simulink model "tanque"  (R2016b)
settings: Solver=ode15s  StartTime=0.0  StopTime=Inf  RelTol=1e-3  EnableMultiTasking=on
libraries: simulink_extras x3
(part 2 of 2)

== system tanque/B 111 ==
  note: Exaustor
  Sinal de entrada : Inport
  Sinal de saída : Outport
  wires:
  Sinal de entrada/1 -> Sinal de saída/1

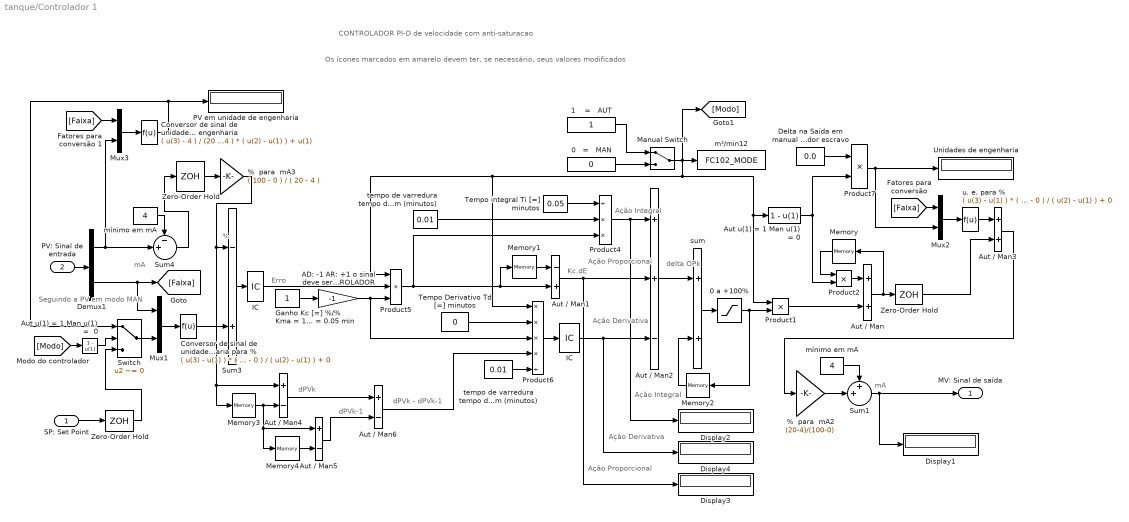
== system tanque/Controlador 1 ==
  note: Ação
      | Derivativa
  note: dPVk - dPVk-1
  note: dPVk
  note: dPVk-1
  note: delta
      | OPk
  note: Ação
      | Integral
  note: Ação
      | Proporcional
  note: Kc.dE
  note: %
  note: mA
  note: CONTROLADOR PI-D de velocidade com anti-saturacao
  note: Os ícones marcados em amarelo devem ter, se necessário, seus valores modificados
  note: Erro
  note: mA
  note: Ação
      | Integral
  note: Ação
      | Derivativa
  note: Ação
      | Proporcional
  note: Seguindo a PV
      | em modo MAN
  SP: Set Point : Inport
  PV: Sinal de entrada : Inport  Port=2
  "  1    =   AUT" : Constant
  " IC" : InitialCondition  Value=0
  %  para  mA2 : Gain  Gain=(20-4)/(100-0)  SaturateOnIntegerOverflow=on  OutDataTypeStr=Inherit: Same as input  ParamDataTypeStr=Inherit: Same as input
  %  para  mA3 : Gain  Gain=( 100 - 0 ) / ( 20 - 4 )  SaturateOnIntegerOverflow=on  OutDataTypeStr=Inherit: Same as input  ParamDataTypeStr=Inherit: Same as input
  0   =   MAN : Constant  Value=0
  0 a +100% : Saturate  UpperLimit=100  LowerLimit=0  LinearizeAsGain=off
  "AD: -1 AR: +1 o sinal deve ser modificado para a correta  AÇÃO  DO  CONTROLADOR " : Gain  Gain=-1  SaturateOnIntegerOverflow=on  OutDataTypeStr=Inherit: Same as input  ParamDataTypeStr=Inherit: Same as input
  Aut / Man : Sum  SaturateOnIntegerOverflow=on  InputSameDT=on  OutDataTypeStr=Inherit: Same as first input
  Aut / Man1 : Sum  Inputs=-+  SaturateOnIntegerOverflow=on  InputSameDT=on  OutDataTypeStr=Inherit: Same as first input
  Aut / Man2 : Sum  Inputs=++-  SaturateOnIntegerOverflow=on  InputSameDT=on  OutDataTypeStr=Inherit: Same as first input
  Aut / Man3 : Sum  SaturateOnIntegerOverflow=on  InputSameDT=on  OutDataTypeStr=Inherit: Same as first input
  Aut / Man4 : Sum  Inputs=+-  SaturateOnIntegerOverflow=on  InputSameDT=on  OutDataTypeStr=Inherit: Same as first input
  Aut / Man5 : Sum  Inputs=+-  SaturateOnIntegerOverflow=on  InputSameDT=on  OutDataTypeStr=Inherit: Same as first input
  Aut / Man6 : Sum  Inputs=+-  SaturateOnIntegerOverflow=on  InputSameDT=on  OutDataTypeStr=Inherit: Same as first input
  Aut u(1) = 1 Man u(1) =  0 : Fcn  Expr=1 - u(1)
  Aut u(1) = 1 Man u(1) = 0 : Fcn  Expr=1 - u(1)
  Conversor de sinal de unidades de engenharia para % : Fcn  Expr=( u(3) - u(1) ) * ( 100 - 0 ) / ( u(2) - u(1) ) + 0
  Conversor de sinal de unidades de  mA  para engenharia : Fcn  Expr=( u(3) - 4 ) / (20 - 4 ) * ( u(2) - u(1) ) + u(1)
  Delta na Saída em manual do controlador [=] unidades de engenharia do SP do controlador escravo : Constant  Value=0.0
  Demux1 : Demux  Outputs=[ 1 2 ]
  Display{1..4} (4 alike) : Display
  Ganho Kc [=] %/% Kma = 1 mA/mA Lambda = 0.05 min : Constant
  IC : InitialCondition  Value=0
  Manual Switch : ManualSwitch
  Memory{,2..4} (4 alike) : Memory  X0=50  InheritSampleTime=on
  Memory1 : Memory  InheritSampleTime=on
  Mux1 : Mux  Inputs=[ 2 1 ]
  Mux2 : Mux  Inputs=[ 2 1 ]
  Mux3 : Mux  Inputs=[ 2 1 ]
  PV em unidade de engenharia : Display
  Product1 : Product  SaturateOnIntegerOverflow=on  RndMeth=Zero  InputSameDT=on  OutDataTypeStr=Inherit: Same as first input
  Product2 : Product  SaturateOnIntegerOverflow=on  RndMeth=Zero  InputSameDT=on  OutDataTypeStr=Inherit: Same as first input
  Product4 : Product  Inputs=/**  SaturateOnIntegerOverflow=on  RndMeth=Zero  InputSameDT=on  OutDataTypeStr=Inherit: Same as first input
  Product5 : Product  Inputs=3  SaturateOnIntegerOverflow=on  RndMeth=Zero  InputSameDT=on  OutDataTypeStr=Inherit: Same as first input
  Product6 : Product  Inputs=****/  SaturateOnIntegerOverflow=on  RndMeth=Zero  InputSameDT=on  OutDataTypeStr=Inherit: Same as first input
  Product7 : Product  SaturateOnIntegerOverflow=on  RndMeth=Zero  InputSameDT=on  OutDataTypeStr=Inherit: Same as first input
  Sum1 : Sum  Inputs=++|  SaturateOnIntegerOverflow=on  InputSameDT=on  OutDataTypeStr=Inherit: Same as first input
  Sum3 : Sum  Inputs=-+  SaturateOnIntegerOverflow=on  InputSameDT=on  OutDataTypeStr=Inherit: Same as first input
  Sum4 : Sum  Inputs=-+|  SaturateOnIntegerOverflow=on  InputSameDT=on  OutDataTypeStr=Inherit: Same as first input
  Switch : Switch  Criteria=u2 ~= 0  RndMeth=Nearest  SaturateOnIntegerOverflow=on
  Tempo Derivativo Td [=] minutos : Constant  Value=0
  Tempo integral Ti [=] minutos : Constant  Value=0.05
  Unidades de engenharia : Display
  Zero-Order Hold : ZeroOrderHold  SampleTime=0.01
  "Zero-Order Hold " : ZeroOrderHold  SampleTime=0.01
  "Zero-Order Hold " : ZeroOrderHold  SampleTime=0.01
  m³/min12 : ToWorkspace  VariableName=FC102_MODE  SampleTime=-1
      settings: Decimation=10
  mínimo em mA : Constant  Value=4
  "mínimo em mA " : Constant  Value=4
  sum : Sum  SaturateOnIntegerOverflow=on  InputSameDT=on  OutDataTypeStr=Inherit: Same as first input
  tempo de varredura tempo de amostragem (minutos) : Constant  Value=0.01
  "tempo de varredura tempo de amostragem (minutos) " : Constant  Value=0.01
  u. e. para % : Fcn  Expr=( u(3) - u(1) ) * ( 100 - 0 ) / ( u(2) - u(1) ) + 0
  MV: Sinal de saída : Outport
  wires:
  "AD: -1 AR: +1 o sinal deve ser modificado para a correta  AÇÃO  DO  CONTROLADOR "/1 -> Product5/3, Product6/3
  " IC"/1 -> Aut / Man2/3, Display4/1
  "tempo de varredura tempo de amostragem (minutos) "/1 -> Product6/5
  Aut / Man5/1 -> Aut / Man6/2
  Aut / Man4/1 -> Aut / Man6/1
  Conversor de sinal de unidades de engenharia para %/1 -> Sum3/2
  Product6/1 -> " IC"/1
  Tempo Derivativo Td [=] minutos/1 -> Product6/2
  Aut / Man6/1 -> Product6/4
  Memory4/1 -> Aut / Man5/2
  Memory3/1 -> Aut / Man4/2, Aut / Man5/1, Memory4/1
  Ganho Kc [=] %/% Kma = 1 mA/mA Lambda = 0.05 min/1 -> "AD: -1 AR: +1 o sinal deve ser modificado para a correta  AÇÃO  DO  CONTROLADOR "/1
  IC/1 -> Product5/2
  0 a +100%/1 -> Product1/2, Memory2/1
  Memory2/1 -> sum/2
  sum/1 -> 0 a +100%/1
  Aut / Man2/1 -> sum/1
  Aut / Man1/1 -> Aut / Man2/2, Display3/1
  Product4/1 -> Aut / Man2/1, Display2/1
  Memory1/1 -> Aut / Man1/1
  Memory/1 -> Product2/1
  Aut / Man/1 -> Memory/1, Zero-Order Hold/1
  Aut u(1) = 1 Man u(1) = 0/1 -> Product2/2, Product7/2
  Product2/1 -> Aut / Man/1
  Product1/1 -> Aut / Man/2
  Product5/1 -> Memory1/1, Aut / Man1/2, Product4/3
  Sum3/1 -> IC/1
  mínimo em mA/1 -> Sum4/1
  Demux1/1 -> Sum4/2, Mux3/2
  Mux1/1 -> Conversor de sinal de unidades de engenharia para %/1
  SP: Set Point/1 -> "Zero-Order Hold "/1
  PV: Sinal de entrada/1 -> Demux1/1
  "mínimo em mA "/1 -> Sum1/1
  Sum1/1 -> MV: Sinal de saída/1, Display1/1
  Sum4/1 -> "Zero-Order Hold "/1
  "Zero-Order Hold "/1 -> %  para  mA3/1
  %  para  mA3/1 -> Memory3/1, Aut / Man4/1, Sum3/1
  Manual Switch/1 -> Aut u(1) = 1 Man u(1) = 0/1, Product1/1, Product5/1, Product6/1, [Modo], m³/min12/1
  Delta na Saída em manual do controlador [=] unidades de engenharia do SP do controlador escravo/1 -> Product7/1
  Product7/1 -> Unidades de engenharia/1, Mux2/2
  Demux1/2 -> Mux1/1, [Faixa]
  "Zero-Order Hold "/1 -> Switch/3
  u. e. para %/1 -> Aut / Man3/1
  Zero-Order Hold/1 -> Aut / Man3/2
  Mux2/1 -> u. e. para %/1
  [Faixa] -> Mux2/1
  Aut / Man3/1 -> %  para  mA2/1
  %  para  mA2/1 -> Sum1/2
  "  1    =   AUT"/1 -> Manual Switch/1
  0   =   MAN/1 -> Manual Switch/2
  [Modo] -> Aut u(1) = 1 Man u(1) =  0/1
  Switch/1 -> Mux1/2
  Aut u(1) = 1 Man u(1) =  0/1 -> Switch/2
  Mux3/1 -> Conversor de sinal de unidades de  mA  para engenharia/1
  [Faixa] -> Mux3/1
  Conversor de sinal de unidades de  mA  para engenharia/1 -> Switch/1, PV em unidade de engenharia/1
  Tempo integral Ti [=] minutos/1 -> Product4/1
  tempo de varredura tempo de amostragem (minutos)/1 -> Product4/2

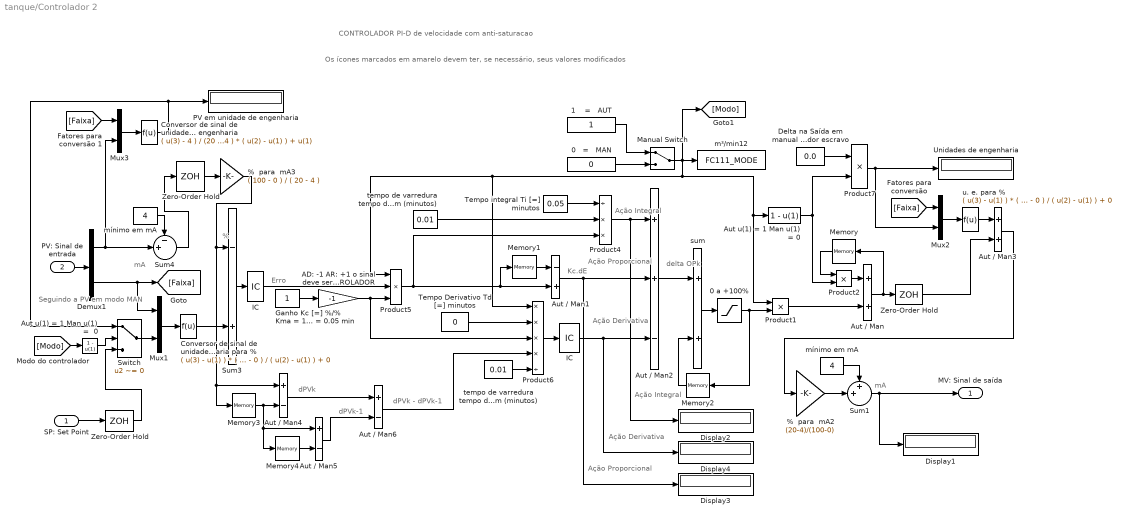
== system tanque/Controlador 2 ==
  note: Ação
      | Derivativa
  note: dPVk - dPVk-1
  note: dPVk
  note: dPVk-1
  note: delta
      | OPk
  note: Ação
      | Integral
  note: Ação
      | Proporcional
  note: Kc.dE
  note: %
  note: mA
  note: CONTROLADOR PI-D de velocidade com anti-saturacao
  note: Os ícones marcados em amarelo devem ter, se necessário, seus valores modificados
  note: Erro
  note: mA
  note: Ação
      | Integral
  note: Ação
      | Derivativa
  note: Ação
      | Proporcional
  note: Seguindo a PV
      | em modo MAN
  SP: Set Point : Inport
  PV: Sinal de entrada : Inport  Port=2
  "  1    =   AUT" : Constant
  " IC" : InitialCondition  Value=0
  %  para  mA2 : Gain  Gain=(20-4)/(100-0)  SaturateOnIntegerOverflow=on  OutDataTypeStr=Inherit: Same as input  ParamDataTypeStr=Inherit: Same as input
  %  para  mA3 : Gain  Gain=( 100 - 0 ) / ( 20 - 4 )  SaturateOnIntegerOverflow=on  OutDataTypeStr=Inherit: Same as input  ParamDataTypeStr=Inherit: Same as input
  0   =   MAN : Constant  Value=0
  0 a +100% : Saturate  UpperLimit=100  LowerLimit=0  LinearizeAsGain=off
  "AD: -1 AR: +1 o sinal deve ser modificado para a correta  AÇÃO  DO  CONTROLADOR " : Gain  Gain=-1  SaturateOnIntegerOverflow=on  OutDataTypeStr=Inherit: Same as input  ParamDataTypeStr=Inherit: Same as input
  Aut / Man : Sum  SaturateOnIntegerOverflow=on  InputSameDT=on  OutDataTypeStr=Inherit: Same as first input
  Aut / Man1 : Sum  Inputs=-+  SaturateOnIntegerOverflow=on  InputSameDT=on  OutDataTypeStr=Inherit: Same as first input
  Aut / Man2 : Sum  Inputs=++-  SaturateOnIntegerOverflow=on  InputSameDT=on  OutDataTypeStr=Inherit: Same as first input
  Aut / Man3 : Sum  SaturateOnIntegerOverflow=on  InputSameDT=on  OutDataTypeStr=Inherit: Same as first input
  Aut / Man4 : Sum  Inputs=+-  SaturateOnIntegerOverflow=on  InputSameDT=on  OutDataTypeStr=Inherit: Same as first input
  Aut / Man5 : Sum  Inputs=+-  SaturateOnIntegerOverflow=on  InputSameDT=on  OutDataTypeStr=Inherit: Same as first input
  Aut / Man6 : Sum  Inputs=+-  SaturateOnIntegerOverflow=on  InputSameDT=on  OutDataTypeStr=Inherit: Same as first input
  Aut u(1) = 1 Man u(1) =  0 : Fcn  Expr=1 - u(1)
  Aut u(1) = 1 Man u(1) = 0 : Fcn  Expr=1 - u(1)
  Conversor de sinal de unidades de engenharia para % : Fcn  Expr=( u(3) - u(1) ) * ( 100 - 0 ) / ( u(2) - u(1) ) + 0
  Conversor de sinal de unidades de  mA  para engenharia : Fcn  Expr=( u(3) - 4 ) / (20 - 4 ) * ( u(2) - u(1) ) + u(1)
  Delta na Saída em manual do controlador [=] unidades de engenharia do SP do controlador escravo : Constant  Value=0.0
  Demux1 : Demux  Outputs=[ 1 2 ]
  Display{1..4} (4 alike) : Display
  Ganho Kc [=] %/% Kma = 1 mA/mA Lambda = 0.05 min : Constant
  IC : InitialCondition  Value=0
  Manual Switch : ManualSwitch
  Memory{,2..4} (4 alike) : Memory  X0=50  InheritSampleTime=on
  Memory1 : Memory  InheritSampleTime=on
  Mux1 : Mux  Inputs=[ 2 1 ]
  Mux2 : Mux  Inputs=[ 2 1 ]
  Mux3 : Mux  Inputs=[ 2 1 ]
  PV em unidade de engenharia : Display
  Product1 : Product  SaturateOnIntegerOverflow=on  RndMeth=Zero  InputSameDT=on  OutDataTypeStr=Inherit: Same as first input
  Product2 : Product  SaturateOnIntegerOverflow=on  RndMeth=Zero  InputSameDT=on  OutDataTypeStr=Inherit: Same as first input
  Product4 : Product  Inputs=/**  SaturateOnIntegerOverflow=on  RndMeth=Zero  InputSameDT=on  OutDataTypeStr=Inherit: Same as first input
  Product5 : Product  Inputs=3  SaturateOnIntegerOverflow=on  RndMeth=Zero  InputSameDT=on  OutDataTypeStr=Inherit: Same as first input
  Product6 : Product  Inputs=****/  SaturateOnIntegerOverflow=on  RndMeth=Zero  InputSameDT=on  OutDataTypeStr=Inherit: Same as first input
  Product7 : Product  SaturateOnIntegerOverflow=on  RndMeth=Zero  InputSameDT=on  OutDataTypeStr=Inherit: Same as first input
  Sum1 : Sum  Inputs=++|  SaturateOnIntegerOverflow=on  InputSameDT=on  OutDataTypeStr=Inherit: Same as first input
  Sum3 : Sum  Inputs=-+  SaturateOnIntegerOverflow=on  InputSameDT=on  OutDataTypeStr=Inherit: Same as first input
  Sum4 : Sum  Inputs=-+|  SaturateOnIntegerOverflow=on  InputSameDT=on  OutDataTypeStr=Inherit: Same as first input
  Switch : Switch  Criteria=u2 ~= 0  RndMeth=Nearest  SaturateOnIntegerOverflow=on
  Tempo Derivativo Td [=] minutos : Constant  Value=0
  Tempo integral Ti [=] minutos : Constant  Value=0.05
  Unidades de engenharia : Display
  Zero-Order Hold : ZeroOrderHold  SampleTime=0.01
  "Zero-Order Hold " : ZeroOrderHold  SampleTime=0.01
  "Zero-Order Hold " : ZeroOrderHold  SampleTime=0.01
  m³/min12 : ToWorkspace  VariableName=FC111_MODE  SampleTime=-1
      settings: Decimation=10
  mínimo em mA : Constant  Value=4
  "mínimo em mA " : Constant  Value=4
  sum : Sum  SaturateOnIntegerOverflow=on  InputSameDT=on  OutDataTypeStr=Inherit: Same as first input
  tempo de varredura tempo de amostragem (minutos) : Constant  Value=0.01
  "tempo de varredura tempo de amostragem (minutos) " : Constant  Value=0.01
  u. e. para % : Fcn  Expr=( u(3) - u(1) ) * ( 100 - 0 ) / ( u(2) - u(1) ) + 0
  MV: Sinal de saída : Outport
  wires:
  "AD: -1 AR: +1 o sinal deve ser modificado para a correta  AÇÃO  DO  CONTROLADOR "/1 -> Product5/3, Product6/3
  " IC"/1 -> Aut / Man2/3, Display4/1
  "tempo de varredura tempo de amostragem (minutos) "/1 -> Product6/5
  Aut / Man5/1 -> Aut / Man6/2
  Aut / Man4/1 -> Aut / Man6/1
  Conversor de sinal de unidades de engenharia para %/1 -> Sum3/2
  Product6/1 -> " IC"/1
  Tempo Derivativo Td [=] minutos/1 -> Product6/2
  Aut / Man6/1 -> Product6/4
  Memory4/1 -> Aut / Man5/2
  Memory3/1 -> Aut / Man4/2, Aut / Man5/1, Memory4/1
  Ganho Kc [=] %/% Kma = 1 mA/mA Lambda = 0.05 min/1 -> "AD: -1 AR: +1 o sinal deve ser modificado para a correta  AÇÃO  DO  CONTROLADOR "/1
  IC/1 -> Product5/2
  0 a +100%/1 -> Product1/2, Memory2/1
  Memory2/1 -> sum/2
  sum/1 -> 0 a +100%/1
  Aut / Man2/1 -> sum/1
  Aut / Man1/1 -> Aut / Man2/2, Display3/1
  Product4/1 -> Aut / Man2/1, Display2/1
  Memory1/1 -> Aut / Man1/1
  Memory/1 -> Product2/1
  Aut / Man/1 -> Memory/1, Zero-Order Hold/1
  Aut u(1) = 1 Man u(1) = 0/1 -> Product2/2, Product7/2
  Product2/1 -> Aut / Man/1
  Product1/1 -> Aut / Man/2
  Product5/1 -> Memory1/1, Aut / Man1/2, Product4/3
  Sum3/1 -> IC/1
  mínimo em mA/1 -> Sum4/1
  Demux1/1 -> Sum4/2, Mux3/2
  Mux1/1 -> Conversor de sinal de unidades de engenharia para %/1
  SP: Set Point/1 -> "Zero-Order Hold "/1
  PV: Sinal de entrada/1 -> Demux1/1
  "mínimo em mA "/1 -> Sum1/1
  Sum1/1 -> MV: Sinal de saída/1, Display1/1
  Sum4/1 -> "Zero-Order Hold "/1
  "Zero-Order Hold "/1 -> %  para  mA3/1
  %  para  mA3/1 -> Memory3/1, Aut / Man4/1, Sum3/1
  Manual Switch/1 -> Aut u(1) = 1 Man u(1) = 0/1, Product1/1, Product5/1, Product6/1, [Modo], m³/min12/1
  Delta na Saída em manual do controlador [=] unidades de engenharia do SP do controlador escravo/1 -> Product7/1
  Product7/1 -> Unidades de engenharia/1, Mux2/2
  Demux1/2 -> Mux1/1, [Faixa]
  "Zero-Order Hold "/1 -> Switch/3
  u. e. para %/1 -> Aut / Man3/1
  Zero-Order Hold/1 -> Aut / Man3/2
  Mux2/1 -> u. e. para %/1
  [Faixa] -> Mux2/1
  Aut / Man3/1 -> %  para  mA2/1
  %  para  mA2/1 -> Sum1/2
  "  1    =   AUT"/1 -> Manual Switch/1
  0   =   MAN/1 -> Manual Switch/2
  [Modo] -> Aut u(1) = 1 Man u(1) =  0/1
  Switch/1 -> Mux1/2
  Aut u(1) = 1 Man u(1) =  0/1 -> Switch/2
  Mux3/1 -> Conversor de sinal de unidades de  mA  para engenharia/1
  [Faixa] -> Mux3/1
  Conversor de sinal de unidades de  mA  para engenharia/1 -> Switch/1, PV em unidade de engenharia/1
  Tempo integral Ti [=] minutos/1 -> Product4/1
  tempo de varredura tempo de amostragem (minutos)/1 -> Product4/2

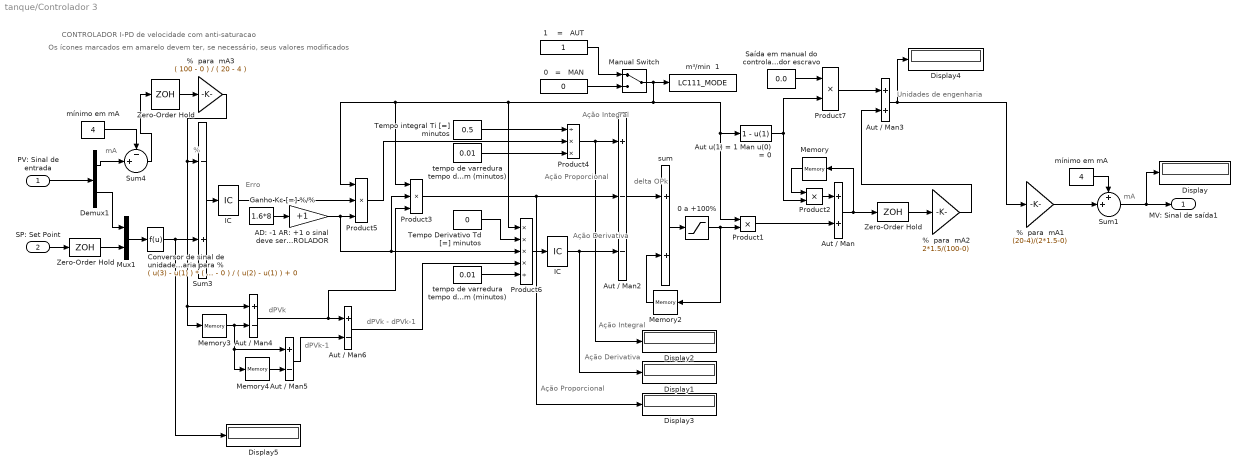
== system tanque/Controlador 3 ==
  note: Erro
  note: Os ícones marcados em amarelo devem ter, se necessário, seus valores modificados
  note: CONTROLADOR I-PD de velocidade com anti-saturacao
  note: mA
  note: %
  note: Ação
      | Proporcional
  note: delta
      | OPk
  note: dPVk-1
  note: dPVk
  note: dPVk - dPVk-1
  note: Ação
      | Derivativa
  note: Ação
      | Integral
  note: Unidades
      | de
      | engenharia
  note: Ação
      | Integral
  note: Ação
      | Derivativa
  note: Ação
      | Proporcional
  note: mA
  PV: Sinal de entrada : Inport
  SP: Set Point : Inport  Port=2
  "   m³/min  1" : ToWorkspace  VariableName=LC111_MODE  SampleTime=-1
      settings: Decimation=10
  "  1    =   AUT" : Constant
  " IC" : InitialCondition  Value=0
  %  para  mA1 : Gain  Gain=(20-4)/(2*1.5-0)  SaturateOnIntegerOverflow=on  OutDataTypeStr=Inherit: Same as input  ParamDataTypeStr=Inherit: Same as input
  %  para  mA2 : Gain  Gain=2*1.5/(100-0)  SaturateOnIntegerOverflow=on  OutDataTypeStr=Inherit: Same as input  ParamDataTypeStr=Inherit: Same as input
  %  para  mA3 : Gain  Gain=( 100 - 0 ) / ( 20 - 4 )  SaturateOnIntegerOverflow=on  OutDataTypeStr=Inherit: Same as input  ParamDataTypeStr=Inherit: Same as input
  0   =   MAN : Constant  Value=0
  0 a +100% : Saturate  UpperLimit=100  LowerLimit=0  LinearizeAsGain=off
  "AD: -1 AR: +1 o sinal deve ser modificado para a correta  AÇÃO  DO  CONTROLADOR " : Gain  Gain=+1  SaturateOnIntegerOverflow=on  OutDataTypeStr=Inherit: Same as input  ParamDataTypeStr=Inherit: Same as input
  Aut / Man : Sum  SaturateOnIntegerOverflow=on  InputSameDT=on  OutDataTypeStr=Inherit: Same as first input
  Aut / Man2 : Sum  Inputs=+--  SaturateOnIntegerOverflow=on  InputSameDT=on  OutDataTypeStr=Inherit: Same as first input
  Aut / Man3 : Sum  SaturateOnIntegerOverflow=on  InputSameDT=on  OutDataTypeStr=Inherit: Same as first input
  Aut / Man4 : Sum  Inputs=+-  SaturateOnIntegerOverflow=on  InputSameDT=on  OutDataTypeStr=Inherit: Same as first input
  Aut / Man5 : Sum  Inputs=+-  SaturateOnIntegerOverflow=on  InputSameDT=on  OutDataTypeStr=Inherit: Same as first input
  Aut / Man6 : Sum  Inputs=+-  SaturateOnIntegerOverflow=on  InputSameDT=on  OutDataTypeStr=Inherit: Same as first input
  Aut u(1) = 1 Man u(0) = 0 : Fcn  Expr=1 - u(1)
  Conversor de sinal de unidades de engenharia para % : Fcn  Expr=( u(3) - u(1) ) * ( 100 - 0 ) / ( u(2) - u(1) ) + 0
  Demux1 : Demux  Outputs=[ 1 2 ]
  Display{,1..5} (6 alike) : Display
  Ganho Kc [=] %/% : Constant  Value=1.6*8
  IC : InitialCondition  Value=0
  Manual Switch : ManualSwitch
  Memory{,2..4} (4 alike) : Memory  X0=50  InheritSampleTime=on
  Mux1 : Mux  Inputs=[ 2 1 ]
  Product1 : Product  SaturateOnIntegerOverflow=on  RndMeth=Zero  InputSameDT=on  OutDataTypeStr=Inherit: Same as first input
  Product2 : Product  SaturateOnIntegerOverflow=on  RndMeth=Zero  InputSameDT=on  OutDataTypeStr=Inherit: Same as first input
  Product3 : Product  Inputs=3  SaturateOnIntegerOverflow=on  RndMeth=Zero  InputSameDT=on  OutDataTypeStr=Inherit: Same as first input
  Product4 : Product  Inputs=/**  SaturateOnIntegerOverflow=on  RndMeth=Zero  InputSameDT=on  OutDataTypeStr=Inherit: Same as first input
  Product5 : Product  Inputs=3  SaturateOnIntegerOverflow=on  RndMeth=Zero  InputSameDT=on  OutDataTypeStr=Inherit: Same as first input
  Product6 : Product  Inputs=****/  SaturateOnIntegerOverflow=on  RndMeth=Zero  InputSameDT=on  OutDataTypeStr=Inherit: Same as first input
  Product7 : Product  SaturateOnIntegerOverflow=on  RndMeth=Zero  InputSameDT=on  OutDataTypeStr=Inherit: Same as first input
  Saída em manual do controlador [=] unidades de engenharia do SP do controlador escravo : Constant  Value=0.0
  Sum1 : Sum  Inputs=++|  SaturateOnIntegerOverflow=on  InputSameDT=on  OutDataTypeStr=Inherit: Same as first input
  Sum3 : Sum  Inputs=-+  SaturateOnIntegerOverflow=on  InputSameDT=on  OutDataTypeStr=Inherit: Same as first input
  Sum4 : Sum  Inputs=-+|  SaturateOnIntegerOverflow=on  InputSameDT=on  OutDataTypeStr=Inherit: Same as first input
  Tempo Derivativo Td [=] minutos : Constant  Value=0
  Tempo integral Ti [=] minutos : Constant  Value=0.5
  Zero-Order Hold : ZeroOrderHold  SampleTime=0.01
  "Zero-Order Hold " : ZeroOrderHold  SampleTime=0.01
  "Zero-Order Hold " : ZeroOrderHold  SampleTime=0.01
  mínimo em mA : Constant  Value=4
  "mínimo em mA " : Constant  Value=4
  sum : Sum  SaturateOnIntegerOverflow=on  InputSameDT=on  OutDataTypeStr=Inherit: Same as first input
  tempo de varredura tempo de amostragem (minutos) : Constant  Value=0.01
  "tempo de varredura tempo de amostragem (minutos) " : Constant  Value=0.01
  MV: Sinal de saída1 : Outport
  wires:
  PV: Sinal de entrada/1 -> Demux1/1
  SP: Set Point/1 -> Zero-Order Hold/1
  %  para  mA3/1 -> Sum3/1, Aut / Man4/1, Memory3/1
  Demux1/1 -> Sum4/2
  mínimo em mA/1 -> Sum4/1
  Sum3/1 -> IC/1
  Product5/1 -> Product4/2
  Manual Switch/1 -> Product1/1, Aut u(1) = 1 Man u(0) = 0/1, Product6/1, Product5/1, Product3/1, "   m³/min  1"/1
  Product1/1 -> Aut / Man/2
  Product2/1 -> Aut / Man/1
  Aut u(1) = 1 Man u(0) = 0/1 -> Product2/2, Product7/2
  Aut / Man/1 -> Memory/1, "Zero-Order Hold "/1
  Memory/1 -> Product2/1
  Tempo integral Ti [=] minutos/1 -> Product4/1
  tempo de varredura tempo de amostragem (minutos)/1 -> Product4/3
  Product4/1 -> Aut / Man2/1, Display2/1
  Aut / Man2/1 -> sum/1
  sum/1 -> 0 a +100%/1
  Memory2/1 -> sum/2
  0 a +100%/1 -> Memory2/1, Product1/2
  IC/1 -> Product5/2
  Ganho Kc [=] %/%/1 -> "AD: -1 AR: +1 o sinal deve ser modificado para a correta  AÇÃO  DO  CONTROLADOR "/1
  Memory3/1 -> Memory4/1, Aut / Man5/1, Aut / Man4/2
  Memory4/1 -> Aut / Man5/2
  Aut / Man6/1 -> Product6/4
  Product6/1 -> " IC"/1
  Conversor de sinal de unidades de engenharia para %/1 -> Sum3/2, Display5/1
  Aut / Man4/1 -> Aut / Man6/1, Product3/3
  Aut / Man5/1 -> Aut / Man6/2
  "tempo de varredura tempo de amostragem (minutos) "/1 -> Product6/5
  " IC"/1 -> Aut / Man2/3, Display1/1
  "AD: -1 AR: +1 o sinal deve ser modificado para a correta  AÇÃO  DO  CONTROLADOR "/1 -> Product6/3, Product3/2, Product5/3
  Product3/1 -> Aut / Man2/2, Display3/1
  "Zero-Order Hold "/1 -> %  para  mA3/1
  Sum4/1 -> "Zero-Order Hold "/1
  "Zero-Order Hold "/1 -> %  para  mA2/1
  Saída em manual do controlador [=] unidades de engenharia do SP do controlador escravo/1 -> Product7/1
  Product7/1 -> Aut / Man3/1
  %  para  mA2/1 -> Aut / Man3/2
  Aut / Man3/1 -> %  para  mA1/1, Display4/1
  Mux1/1 -> Conversor de sinal de unidades de engenharia para %/1
  Demux1/2 -> Mux1/1
  Zero-Order Hold/1 -> Mux1/2
  "  1    =   AUT"/1 -> Manual Switch/1
  0   =   MAN/1 -> Manual Switch/2
  Tempo Derivativo Td [=] minutos/1 -> Product6/2
  "mínimo em mA "/1 -> Sum1/1
  %  para  mA1/1 -> Sum1/2
  Sum1/1 -> Display/1, MV: Sinal de saída1/1

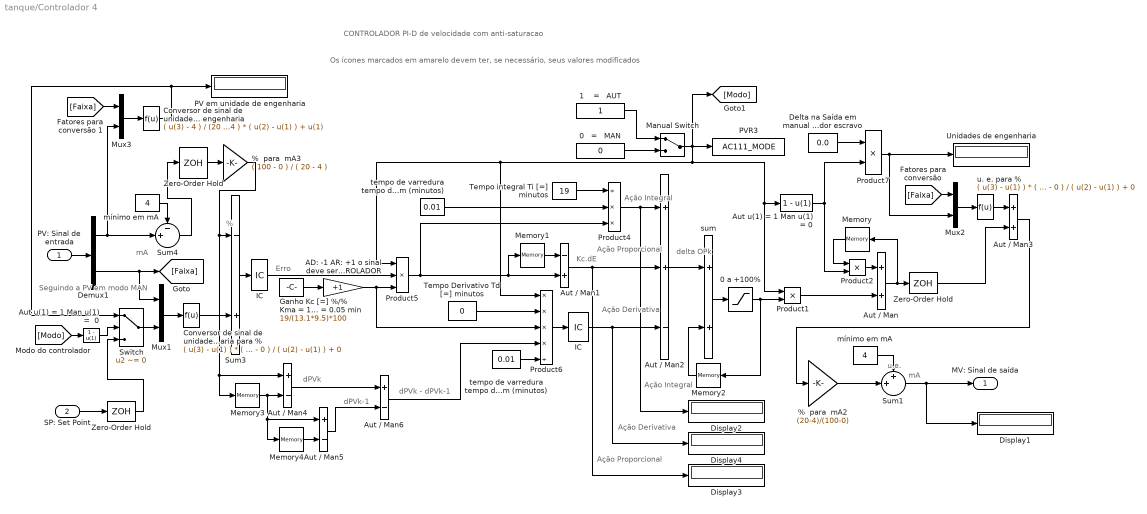
== system tanque/Controlador 4 ==
  note: Ação
      | Derivativa
  note: dPVk - dPVk-1
  note: dPVk
  note: dPVk-1
  note: delta
      | OPk
  note: Ação
      | Integral
  note: Ação
      | Proporcional
  note: Kc.dE
  note: %
  note: mA
  note: CONTROLADOR PI-D de velocidade com anti-saturacao
  note: Os ícones marcados em amarelo devem ter, se necessário, seus valores modificados
  note: Erro
  note: u.e.
  note: Ação
      | Integral
  note: Ação
      | Derivativa
  note: Ação
      | Proporcional
  note: Seguindo a PV
      | em modo MAN
  note: mA
  PV: Sinal de entrada : Inport
  SP: Set Point : Inport  Port=2
  "  1    =   AUT" : Constant
  " IC" : InitialCondition  Value=0
  %  para  mA2 : Gain  Gain=(20-4)/(100-0)  SaturateOnIntegerOverflow=on  OutDataTypeStr=Inherit: Same as input  ParamDataTypeStr=Inherit: Same as input
  %  para  mA3 : Gain  Gain=( 100 - 0 ) / ( 20 - 4 )  SaturateOnIntegerOverflow=on  OutDataTypeStr=Inherit: Same as input  ParamDataTypeStr=Inherit: Same as input
  0   =   MAN : Constant  Value=0
  0 a +100% : Saturate  UpperLimit=100  LowerLimit=0  LinearizeAsGain=off
  "AD: -1 AR: +1 o sinal deve ser modificado para a correta  AÇÃO  DO  CONTROLADOR " : Gain  Gain=+1  SaturateOnIntegerOverflow=on  OutDataTypeStr=Inherit: Same as input  ParamDataTypeStr=Inherit: Same as input
  Aut / Man : Sum  SaturateOnIntegerOverflow=on  InputSameDT=on  OutDataTypeStr=Inherit: Same as first input
  Aut / Man1 : Sum  Inputs=-+  SaturateOnIntegerOverflow=on  InputSameDT=on  OutDataTypeStr=Inherit: Same as first input
  Aut / Man2 : Sum  Inputs=++-  SaturateOnIntegerOverflow=on  InputSameDT=on  OutDataTypeStr=Inherit: Same as first input
  Aut / Man3 : Sum  SaturateOnIntegerOverflow=on  InputSameDT=on  OutDataTypeStr=Inherit: Same as first input
  Aut / Man4 : Sum  Inputs=+-  SaturateOnIntegerOverflow=on  InputSameDT=on  OutDataTypeStr=Inherit: Same as first input
  Aut / Man5 : Sum  Inputs=+-  SaturateOnIntegerOverflow=on  InputSameDT=on  OutDataTypeStr=Inherit: Same as first input
  Aut / Man6 : Sum  Inputs=+-  SaturateOnIntegerOverflow=on  InputSameDT=on  OutDataTypeStr=Inherit: Same as first input
  Aut u(1) = 1 Man u(1) =  0 : Fcn  Expr=1 - u(1)
  Aut u(1) = 1 Man u(1) = 0 : Fcn  Expr=1 - u(1)
  Conversor de sinal de unidades de engenharia para % : Fcn  Expr=( u(3) - u(1) ) * ( 100 - 0 ) / ( u(2) - u(1) ) + 0
  Conversor de sinal de unidades de  mA  para engenharia : Fcn  Expr=( u(3) - 4 ) / (20 - 4 ) * ( u(2) - u(1) ) + u(1)
  Delta na Saída em manual do controlador [=] unidades de engenharia do SP do controlador escravo : Constant  Value=0.0
  Demux1 : Demux  Outputs=[ 1 2 ]
  Display{1..4} (4 alike) : Display
  Ganho Kc [=] %/% Kma = 1 mA/mA Lambda = 0.05 min : Constant  Value=19/(13.1*9.5)*100
  IC : InitialCondition  Value=0
  Manual Switch : ManualSwitch
  Memory{,2..4} (4 alike) : Memory  X0=50  InheritSampleTime=on
  Memory1 : Memory  InheritSampleTime=on
  Mux1 : Mux  Inputs=[ 2 1 ]
  Mux2 : Mux  Inputs=[ 2 1 ]
  Mux3 : Mux  Inputs=[ 2 1 ]
  PV em unidade de engenharia : Display
  PVR3 : ToWorkspace  VariableName=AC111_MODE  SampleTime=-1
      settings: Decimation=10
  Product1 : Product  SaturateOnIntegerOverflow=on  RndMeth=Zero  InputSameDT=on  OutDataTypeStr=Inherit: Same as first input
  Product2 : Product  SaturateOnIntegerOverflow=on  RndMeth=Zero  InputSameDT=on  OutDataTypeStr=Inherit: Same as first input
  Product4 : Product  Inputs=/**  SaturateOnIntegerOverflow=on  RndMeth=Zero  InputSameDT=on  OutDataTypeStr=Inherit: Same as first input
  Product5 : Product  Inputs=3  SaturateOnIntegerOverflow=on  RndMeth=Zero  InputSameDT=on  OutDataTypeStr=Inherit: Same as first input
  Product6 : Product  Inputs=****/  SaturateOnIntegerOverflow=on  RndMeth=Zero  InputSameDT=on  OutDataTypeStr=Inherit: Same as first input
  Product7 : Product  SaturateOnIntegerOverflow=on  RndMeth=Zero  InputSameDT=on  OutDataTypeStr=Inherit: Same as first input
  Sum1 : Sum  Inputs=++|  SaturateOnIntegerOverflow=on  InputSameDT=on  OutDataTypeStr=Inherit: Same as first input
  Sum3 : Sum  Inputs=-+  SaturateOnIntegerOverflow=on  InputSameDT=on  OutDataTypeStr=Inherit: Same as first input
  Sum4 : Sum  Inputs=-+|  SaturateOnIntegerOverflow=on  InputSameDT=on  OutDataTypeStr=Inherit: Same as first input
  Switch : Switch  Criteria=u2 ~= 0  RndMeth=Nearest  SaturateOnIntegerOverflow=on
  Tempo Derivativo Td [=] minutos : Constant  Value=0
  Tempo integral Ti [=] minutos : Constant  Value=19
  Unidades de engenharia : Display
  Zero-Order Hold : ZeroOrderHold  SampleTime=0.01
  "Zero-Order Hold " : ZeroOrderHold  SampleTime=0.01
  "Zero-Order Hold " : ZeroOrderHold  SampleTime=0.01
  mínimo em mA : Constant  Value=4
  "mínimo em mA " : Constant  Value=4
  sum : Sum  SaturateOnIntegerOverflow=on  InputSameDT=on  OutDataTypeStr=Inherit: Same as first input
  tempo de varredura tempo de amostragem (minutos) : Constant  Value=0.01
  "tempo de varredura tempo de amostragem (minutos) " : Constant  Value=0.01
  u. e. para % : Fcn  Expr=( u(3) - u(1) ) * ( 100 - 0 ) / ( u(2) - u(1) ) + 0
  MV: Sinal de saída : Outport
  wires:
  "AD: -1 AR: +1 o sinal deve ser modificado para a correta  AÇÃO  DO  CONTROLADOR "/1 -> Product5/3, Product6/3
  " IC"/1 -> Aut / Man2/3, Display4/1
  "tempo de varredura tempo de amostragem (minutos) "/1 -> Product6/5
  Aut / Man5/1 -> Aut / Man6/2
  Aut / Man4/1 -> Aut / Man6/1
  Conversor de sinal de unidades de engenharia para %/1 -> Sum3/2
  Product6/1 -> " IC"/1
  Tempo Derivativo Td [=] minutos/1 -> Product6/2
  Aut / Man6/1 -> Product6/4
  Memory4/1 -> Aut / Man5/2
  Memory3/1 -> Aut / Man4/2, Aut / Man5/1, Memory4/1
  Ganho Kc [=] %/% Kma = 1 mA/mA Lambda = 0.05 min/1 -> "AD: -1 AR: +1 o sinal deve ser modificado para a correta  AÇÃO  DO  CONTROLADOR "/1
  IC/1 -> Product5/2
  0 a +100%/1 -> Product1/2, Memory2/1
  Memory2/1 -> sum/2
  sum/1 -> 0 a +100%/1
  Aut / Man2/1 -> sum/1
  Aut / Man1/1 -> Aut / Man2/2, Display3/1
  Product4/1 -> Aut / Man2/1, Display2/1
  Memory1/1 -> Aut / Man1/1
  Memory/1 -> Product2/1
  Aut / Man/1 -> Memory/1, Zero-Order Hold/1
  Aut u(1) = 1 Man u(1) = 0/1 -> Product2/2, Product7/2
  Product2/1 -> Aut / Man/1
  Product1/1 -> Aut / Man/2
  Product5/1 -> Memory1/1, Aut / Man1/2, Product4/3
  Sum3/1 -> IC/1
  mínimo em mA/1 -> Sum4/1
  Demux1/1 -> Sum4/2, Mux3/2
  Mux1/1 -> Conversor de sinal de unidades de engenharia para %/1
  SP: Set Point/1 -> "Zero-Order Hold "/1
  PV: Sinal de entrada/1 -> Demux1/1
  Sum4/1 -> "Zero-Order Hold "/1
  "Zero-Order Hold "/1 -> %  para  mA3/1
  %  para  mA3/1 -> Memory3/1, Aut / Man4/1, Sum3/1
  Manual Switch/1 -> Aut u(1) = 1 Man u(1) = 0/1, Product1/1, Product5/1, Product6/1, [Modo], PVR3/1
  Delta na Saída em manual do controlador [=] unidades de engenharia do SP do controlador escravo/1 -> Product7/1
  Product7/1 -> Unidades de engenharia/1, Mux2/2
  Demux1/2 -> Mux1/1, [Faixa]
  "Zero-Order Hold "/1 -> Switch/3
  u. e. para %/1 -> Aut / Man3/1
  Zero-Order Hold/1 -> Aut / Man3/2
  Mux2/1 -> u. e. para %/1
  [Faixa] -> Mux2/1
  Aut / Man3/1 -> %  para  mA2/1
  "  1    =   AUT"/1 -> Manual Switch/1
  0   =   MAN/1 -> Manual Switch/2
  [Modo] -> Aut u(1) = 1 Man u(1) =  0/1
  Switch/1 -> Mux1/2
  Aut u(1) = 1 Man u(1) =  0/1 -> Switch/2
  Mux3/1 -> Conversor de sinal de unidades de  mA  para engenharia/1
  [Faixa] -> Mux3/1
  Conversor de sinal de unidades de  mA  para engenharia/1 -> Switch/1, PV em unidade de engenharia/1
  Tempo integral Ti [=] minutos/1 -> Product4/1
  tempo de varredura tempo de amostragem (minutos)/1 -> Product4/2
  "mínimo em mA "/1 -> Sum1/1
  %  para  mA2/1 -> Sum1/2
  Sum1/1 -> Display1/1, MV: Sinal de saída/1

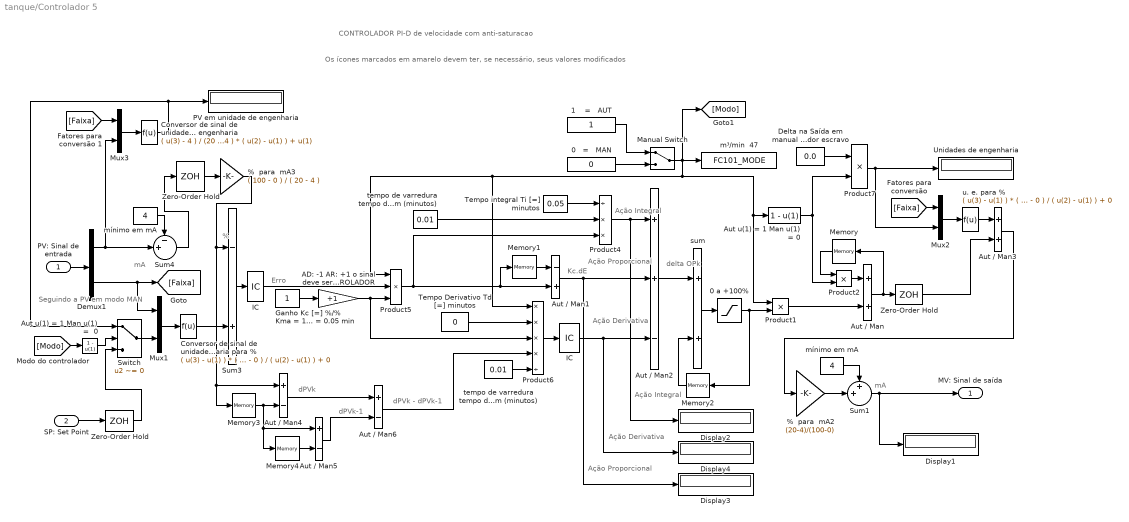
== system tanque/Controlador 5 ==
  note: Ação
      | Derivativa
  note: dPVk - dPVk-1
  note: dPVk
  note: dPVk-1
  note: delta
      | OPk
  note: Ação
      | Integral
  note: Ação
      | Proporcional
  note: Kc.dE
  note: %
  note: mA
  note: CONTROLADOR PI-D de velocidade com anti-saturacao
  note: Os ícones marcados em amarelo devem ter, se necessário, seus valores modificados
  note: Erro
  note: mA
  note: Ação
      | Integral
  note: Ação
      | Derivativa
  note: Ação
      | Proporcional
  note: Seguindo a PV
      | em modo MAN
  PV: Sinal de entrada : Inport
  SP: Set Point : Inport  Port=2
  "   m³/min  47" : ToWorkspace  VariableName=FC101_MODE  SampleTime=-1
      settings: Decimation=10
  "  1    =   AUT" : Constant
  " IC" : InitialCondition  Value=0
  %  para  mA2 : Gain  Gain=(20-4)/(100-0)  SaturateOnIntegerOverflow=on  OutDataTypeStr=Inherit: Same as input  ParamDataTypeStr=Inherit: Same as input
  %  para  mA3 : Gain  Gain=( 100 - 0 ) / ( 20 - 4 )  SaturateOnIntegerOverflow=on  OutDataTypeStr=Inherit: Same as input  ParamDataTypeStr=Inherit: Same as input
  0   =   MAN : Constant  Value=0
  0 a +100% : Saturate  UpperLimit=100  LowerLimit=0  LinearizeAsGain=off
  "AD: -1 AR: +1 o sinal deve ser modificado para a correta  AÇÃO  DO  CONTROLADOR " : Gain  Gain=+1  SaturateOnIntegerOverflow=on  OutDataTypeStr=Inherit: Same as input  ParamDataTypeStr=Inherit: Same as input
  Aut / Man : Sum  SaturateOnIntegerOverflow=on  InputSameDT=on  OutDataTypeStr=Inherit: Same as first input
  Aut / Man1 : Sum  Inputs=-+  SaturateOnIntegerOverflow=on  InputSameDT=on  OutDataTypeStr=Inherit: Same as first input
  Aut / Man2 : Sum  Inputs=++-  SaturateOnIntegerOverflow=on  InputSameDT=on  OutDataTypeStr=Inherit: Same as first input
  Aut / Man3 : Sum  SaturateOnIntegerOverflow=on  InputSameDT=on  OutDataTypeStr=Inherit: Same as first input
  Aut / Man4 : Sum  Inputs=+-  SaturateOnIntegerOverflow=on  InputSameDT=on  OutDataTypeStr=Inherit: Same as first input
  Aut / Man5 : Sum  Inputs=+-  SaturateOnIntegerOverflow=on  InputSameDT=on  OutDataTypeStr=Inherit: Same as first input
  Aut / Man6 : Sum  Inputs=+-  SaturateOnIntegerOverflow=on  InputSameDT=on  OutDataTypeStr=Inherit: Same as first input
  Aut u(1) = 1 Man u(1) =  0 : Fcn  Expr=1 - u(1)
  Aut u(1) = 1 Man u(1) = 0 : Fcn  Expr=1 - u(1)
  Conversor de sinal de unidades de engenharia para % : Fcn  Expr=( u(3) - u(1) ) * ( 100 - 0 ) / ( u(2) - u(1) ) + 0
  Conversor de sinal de unidades de  mA  para engenharia : Fcn  Expr=( u(3) - 4 ) / (20 - 4 ) * ( u(2) - u(1) ) + u(1)
  Delta na Saída em manual do controlador [=] unidades de engenharia do SP do controlador escravo : Constant  Value=0.0
  Demux1 : Demux  Outputs=[ 1 2 ]
  Display{1..4} (4 alike) : Display
  Ganho Kc [=] %/% Kma = 1 mA/mA Lambda = 0.05 min : Constant
  IC : InitialCondition  Value=0
  Manual Switch : ManualSwitch
  Memory{,2..4} (4 alike) : Memory  X0=50  InheritSampleTime=on
  Memory1 : Memory  InheritSampleTime=on
  Mux1 : Mux  Inputs=[ 2 1 ]
  Mux2 : Mux  Inputs=[ 2 1 ]
  Mux3 : Mux  Inputs=[ 2 1 ]
  PV em unidade de engenharia : Display
  Product1 : Product  SaturateOnIntegerOverflow=on  RndMeth=Zero  InputSameDT=on  OutDataTypeStr=Inherit: Same as first input
  Product2 : Product  SaturateOnIntegerOverflow=on  RndMeth=Zero  InputSameDT=on  OutDataTypeStr=Inherit: Same as first input
  Product4 : Product  Inputs=/**  SaturateOnIntegerOverflow=on  RndMeth=Zero  InputSameDT=on  OutDataTypeStr=Inherit: Same as first input
  Product5 : Product  Inputs=3  SaturateOnIntegerOverflow=on  RndMeth=Zero  InputSameDT=on  OutDataTypeStr=Inherit: Same as first input
  Product6 : Product  Inputs=****/  SaturateOnIntegerOverflow=on  RndMeth=Zero  InputSameDT=on  OutDataTypeStr=Inherit: Same as first input
  Product7 : Product  SaturateOnIntegerOverflow=on  RndMeth=Zero  InputSameDT=on  OutDataTypeStr=Inherit: Same as first input
  Sum1 : Sum  Inputs=++|  SaturateOnIntegerOverflow=on  InputSameDT=on  OutDataTypeStr=Inherit: Same as first input
  Sum3 : Sum  Inputs=-+  SaturateOnIntegerOverflow=on  InputSameDT=on  OutDataTypeStr=Inherit: Same as first input
  Sum4 : Sum  Inputs=-+|  SaturateOnIntegerOverflow=on  InputSameDT=on  OutDataTypeStr=Inherit: Same as first input
  Switch : Switch  Criteria=u2 ~= 0  RndMeth=Nearest  SaturateOnIntegerOverflow=on
  Tempo Derivativo Td [=] minutos : Constant  Value=0
  Tempo integral Ti [=] minutos : Constant  Value=0.05
  Unidades de engenharia : Display
  Zero-Order Hold : ZeroOrderHold  SampleTime=0.01
  "Zero-Order Hold " : ZeroOrderHold  SampleTime=0.01
  "Zero-Order Hold " : ZeroOrderHold  SampleTime=0.01
  mínimo em mA : Constant  Value=4
  "mínimo em mA " : Constant  Value=4
  sum : Sum  SaturateOnIntegerOverflow=on  InputSameDT=on  OutDataTypeStr=Inherit: Same as first input
  tempo de varredura tempo de amostragem (minutos) : Constant  Value=0.01
  "tempo de varredura tempo de amostragem (minutos) " : Constant  Value=0.01
  u. e. para % : Fcn  Expr=( u(3) - u(1) ) * ( 100 - 0 ) / ( u(2) - u(1) ) + 0
  MV: Sinal de saída : Outport
  wires:
  "AD: -1 AR: +1 o sinal deve ser modificado para a correta  AÇÃO  DO  CONTROLADOR "/1 -> Product5/3, Product6/3
  " IC"/1 -> Aut / Man2/3, Display4/1
  "tempo de varredura tempo de amostragem (minutos) "/1 -> Product6/5
  Aut / Man5/1 -> Aut / Man6/2
  Aut / Man4/1 -> Aut / Man6/1
  Conversor de sinal de unidades de engenharia para %/1 -> Sum3/2
  Product6/1 -> " IC"/1
  Tempo Derivativo Td [=] minutos/1 -> Product6/2
  Aut / Man6/1 -> Product6/4
  Memory4/1 -> Aut / Man5/2
  Memory3/1 -> Aut / Man4/2, Aut / Man5/1, Memory4/1
  Ganho Kc [=] %/% Kma = 1 mA/mA Lambda = 0.05 min/1 -> "AD: -1 AR: +1 o sinal deve ser modificado para a correta  AÇÃO  DO  CONTROLADOR "/1
  IC/1 -> Product5/2
  0 a +100%/1 -> Product1/2, Memory2/1
  Memory2/1 -> sum/2
  sum/1 -> 0 a +100%/1
  Aut / Man2/1 -> sum/1
  Aut / Man1/1 -> Aut / Man2/2, Display3/1
  Product4/1 -> Aut / Man2/1, Display2/1
  Memory1/1 -> Aut / Man1/1
  Memory/1 -> Product2/1
  Aut / Man/1 -> Memory/1, Zero-Order Hold/1
  Aut u(1) = 1 Man u(1) = 0/1 -> Product2/2, Product7/2
  Product2/1 -> Aut / Man/1
  Product1/1 -> Aut / Man/2
  Product5/1 -> Memory1/1, Aut / Man1/2, Product4/3
  Sum3/1 -> IC/1
  mínimo em mA/1 -> Sum4/1
  Demux1/1 -> Sum4/2, Mux3/2
  Mux1/1 -> Conversor de sinal de unidades de engenharia para %/1
  SP: Set Point/1 -> "Zero-Order Hold "/1
  PV: Sinal de entrada/1 -> Demux1/1
  "mínimo em mA "/1 -> Sum1/1
  Sum1/1 -> MV: Sinal de saída/1, Display1/1
  Sum4/1 -> "Zero-Order Hold "/1
  "Zero-Order Hold "/1 -> %  para  mA3/1
  %  para  mA3/1 -> Memory3/1, Aut / Man4/1, Sum3/1
  Manual Switch/1 -> Aut u(1) = 1 Man u(1) = 0/1, Product1/1, Product5/1, Product6/1, [Modo], "   m³/min  47"/1
  Delta na Saída em manual do controlador [=] unidades de engenharia do SP do controlador escravo/1 -> Product7/1
  Product7/1 -> Unidades de engenharia/1, Mux2/2
  Demux1/2 -> Mux1/1, [Faixa]
  "Zero-Order Hold "/1 -> Switch/3
  u. e. para %/1 -> Aut / Man3/1
  Zero-Order Hold/1 -> Aut / Man3/2
  Mux2/1 -> u. e. para %/1
  [Faixa] -> Mux2/1
  Aut / Man3/1 -> %  para  mA2/1
  %  para  mA2/1 -> Sum1/2
  "  1    =   AUT"/1 -> Manual Switch/1
  0   =   MAN/1 -> Manual Switch/2
  [Modo] -> Aut u(1) = 1 Man u(1) =  0/1
  Switch/1 -> Mux1/2
  Aut u(1) = 1 Man u(1) =  0/1 -> Switch/2
  Mux3/1 -> Conversor de sinal de unidades de  mA  para engenharia/1
  [Faixa] -> Mux3/1
  Conversor de sinal de unidades de  mA  para engenharia/1 -> Switch/1, PV em unidade de engenharia/1
  Tempo integral Ti [=] minutos/1 -> Product4/1
  tempo de varredura tempo de amostragem (minutos)/1 -> Product4/2

== system tanque/FE 101 ==
  note: Placa de orifício
  In1 : Inport
  Out2 : Outport
  wires:
  In1/1 -> Out2/1

== system tanque/FE 102 ==
  note: Placa de orifício
  In1 : Inport
  Out2 : Outport
  Out1 : Outport  Port=2
  wires:
  In1/1 -> Out1/1, Out2/1

== system tanque/FE 111 ==
  note: C
  note: F
  note: Placa de orifício
  In1 : Inport
  Demux26 : Demux  Outputs=2
  Terminator1 : Terminator
  Out1 : Outport
  Out2 : Outport  Port=2
  wires:
  In1/1 -> Out2/1, Demux26/1
  Demux26/1 -> Out1/1
  Demux26/2 -> Terminator1/1

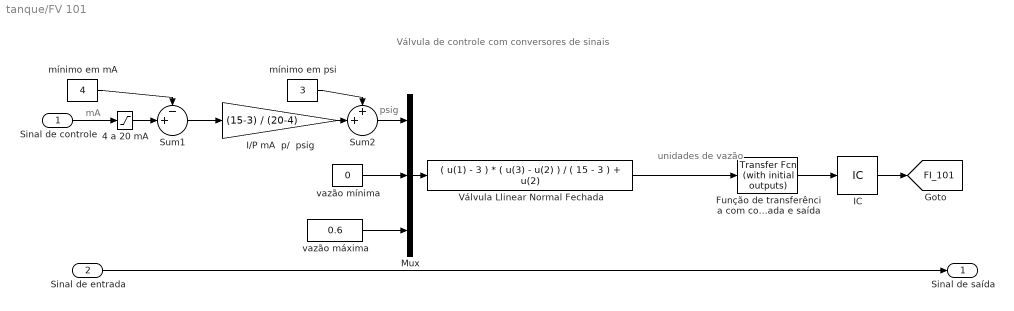
== system tanque/FV 101 ==
  note: psig
  note: unidades
      | de vazão
  note: Válvula de controle com conversores de sinais
  note: mA
  Sinal de controle : Inport
  Sinal de entrada : Inport  Port=2
  4 a 20 mA : Saturate  UpperLimit=20  LowerLimit=4
  Função de transferência com condição inicial na entrada e saída : simulink_extras/Additional Linear/Transfer Fcn (with initial outputs)  N=[1]  D="[ 0.05   1 ]"  Y0=0.2  U0=0.2
  I/P mA  p/  psig : Gain  Gain=(15-3) / (20-4)  SaturateOnIntegerOverflow=on  OutDataTypeStr=Inherit: Same as input  ParamDataTypeStr=Inherit: Same as input
  IC : InitialCondition  Value=0.2
  Mux : Mux  Inputs=3
  Sum1 : Sum  Inputs=-+|  SaturateOnIntegerOverflow=on  InputSameDT=on  OutDataTypeStr=Inherit: Same as first input
  Sum2 : Sum  Inputs=++|  SaturateOnIntegerOverflow=on  InputSameDT=on  OutDataTypeStr=Inherit: Same as first input
  Válvula Llinear Normal Fechada : Fcn  Expr="(  u(1) - 3 ) * ( u(3) - u(2) ) / ( 15 - 3 ) + u(2)"
  mínimo em mA : Constant  Value=4
  mínimo em psi : Constant  Value=3
  vazão máxima : Constant  Value=0.6
  vazão mínima : Constant  Value=0
  Sinal de saída : Outport
  tag scope: FI_101=global
  wires:
  Função de transferência com condição inicial na entrada e saída/1 -> IC/1
  Válvula Llinear Normal Fechada/1 -> Função de transferência com condição inicial na entrada e saída/1
  mínimo em psi/1 -> Sum2/1
  Sum2/1 -> Mux/1
  I/P mA  p/  psig/1 -> Sum2/2
  Sinal de controle/1 -> 4 a 20 mA/1
  Sum1/1 -> I/P mA  p/  psig/1
  mínimo em mA/1 -> Sum1/1
  Mux/1 -> Válvula Llinear Normal Fechada/1
  vazão mínima/1 -> Mux/2
  vazão máxima/1 -> Mux/3
  Sinal de entrada/1 -> Sinal de saída/1
  4 a 20 mA/1 -> Sum1/2
  IC/1 -> [FI_101]

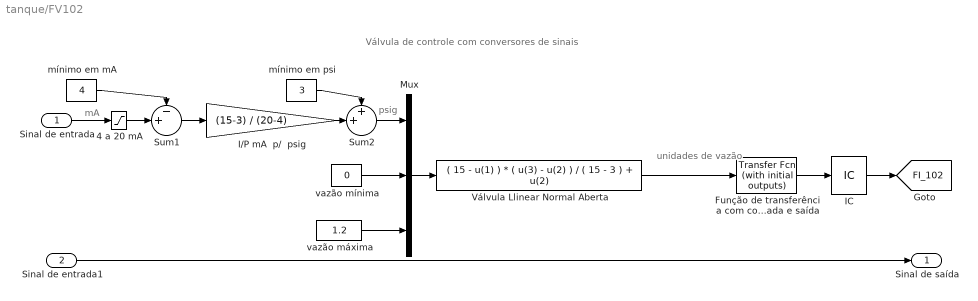
== system tanque/FV102 ==
  note: mA
  note: Válvula de controle com conversores de sinais
  note: unidades
      | de vazão
  note: psig
  Sinal de entrada : Inport
  Sinal de entrada1 : Inport  Port=2
  4 a 20 mA : Saturate  UpperLimit=20  LowerLimit=4
  Função de transferência com condição inicial na entrada e saída : simulink_extras/Additional Linear/Transfer Fcn (with initial outputs)  N=[1]  D="[ 0.05   1 ]"  Y0=0.2  U0=0.2
  I/P mA  p/  psig : Gain  Gain=(15-3) / (20-4)  SaturateOnIntegerOverflow=on  OutDataTypeStr=Inherit: Same as input  ParamDataTypeStr=Inherit: Same as input
  IC : InitialCondition  Value=0
  Mux : Mux  Inputs=3
  Sum1 : Sum  Inputs=-+|  SaturateOnIntegerOverflow=on  InputSameDT=on  OutDataTypeStr=Inherit: Same as first input
  Sum2 : Sum  Inputs=++|  SaturateOnIntegerOverflow=on  InputSameDT=on  OutDataTypeStr=Inherit: Same as first input
  Válvula Llinear Normal Aberta : Fcn  Expr=( 15 - u(1) ) * ( u(3) - u(2) ) / ( 15 - 3 ) + u(2)
  mínimo em mA : Constant  Value=4
  mínimo em psi : Constant  Value=3
  vazão máxima : Constant  Value=1.2
  vazão mínima : Constant  Value=0
  Sinal de saída : Outport
  tag scope: FI_102=global
  wires:
  vazão máxima/1 -> Mux/3
  vazão mínima/1 -> Mux/2
  Mux/1 -> Válvula Llinear Normal Aberta/1
  mínimo em mA/1 -> Sum1/1
  Sum1/1 -> I/P mA  p/  psig/1
  Sinal de entrada/1 -> 4 a 20 mA/1
  I/P mA  p/  psig/1 -> Sum2/2
  Sum2/1 -> Mux/1
  mínimo em psi/1 -> Sum2/1
  Válvula Llinear Normal Aberta/1 -> Função de transferência com condição inicial na entrada e saída/1
  Função de transferência com condição inicial na entrada e saída/1 -> IC/1
  Sinal de entrada1/1 -> Sinal de saída/1
  IC/1 -> [FI_102]
  4 a 20 mA/1 -> Sum1/2

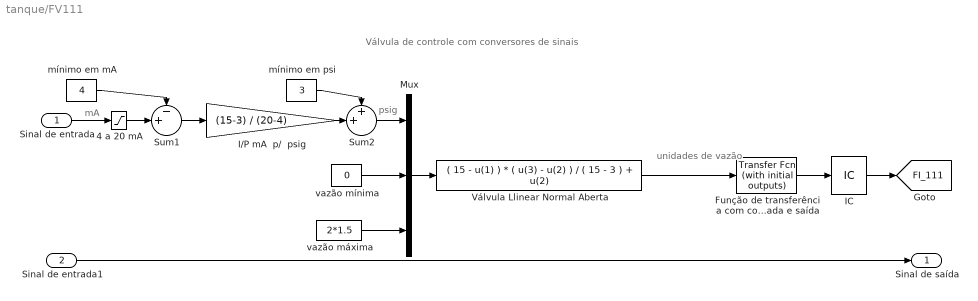
== system tanque/FV111 ==
  note: mA
  note: Válvula de controle com conversores de sinais
  note: unidades
      | de vazão
  note: psig
  Sinal de entrada : Inport
  Sinal de entrada1 : Inport  Port=2
  4 a 20 mA : Saturate  UpperLimit=20  LowerLimit=4
  Função de transferência com condição inicial na entrada e saída : simulink_extras/Additional Linear/Transfer Fcn (with initial outputs)  N=[1]  D="[ 0.05   1 ]"  Y0=0.2  U0=0.2
  I/P mA  p/  psig : Gain  Gain=(15-3) / (20-4)  SaturateOnIntegerOverflow=on  OutDataTypeStr=Inherit: Same as input  ParamDataTypeStr=Inherit: Same as input
  IC : InitialCondition  Value=0.2
  Mux : Mux  Inputs=3
  Sum1 : Sum  Inputs=-+|  SaturateOnIntegerOverflow=on  InputSameDT=on  OutDataTypeStr=Inherit: Same as first input
  Sum2 : Sum  Inputs=++|  SaturateOnIntegerOverflow=on  InputSameDT=on  OutDataTypeStr=Inherit: Same as first input
  Válvula Llinear Normal Aberta : Fcn  Expr=( 15 - u(1) ) * ( u(3) - u(2) ) / ( 15 - 3 ) + u(2)
  mínimo em mA : Constant  Value=4
  mínimo em psi : Constant  Value=3
  vazão máxima : Constant  Value=2*1.5
  vazão mínima : Constant  Value=0
  Sinal de saída : Outport
  tag scope: FI_111=global
  wires:
  vazão máxima/1 -> Mux/3
  vazão mínima/1 -> Mux/2
  Mux/1 -> Válvula Llinear Normal Aberta/1
  mínimo em mA/1 -> Sum1/1
  Sum1/1 -> I/P mA  p/  psig/1
  Sinal de entrada/1 -> 4 a 20 mA/1
  I/P mA  p/  psig/1 -> Sum2/2
  Sum2/1 -> Mux/1
  mínimo em psi/1 -> Sum2/1
  Válvula Llinear Normal Aberta/1 -> Função de transferência com condição inicial na entrada e saída/1
  Função de transferência com condição inicial na entrada e saída/1 -> IC/1
  Sinal de entrada1/1 -> Sinal de saída/1
  IC/1 -> [FI_111]
  4 a 20 mA/1 -> Sum1/2

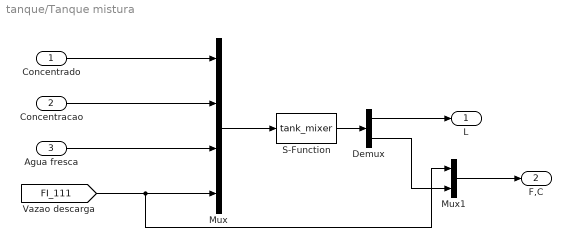
== system tanque/Tanque mistura ==
  Concentrado : Inport
  Concentracao : Inport  Port=2
  Agua fresca : Inport  Port=3
  Demux : Demux  Outputs=2
  Mux : Mux
  Mux1 : Mux  Inputs=2
  S-Function : S-Function  FunctionName=tank_mixer  SFunctionDeploymentMode=off  EnableBusSupport=off
  L : Outport
  F,C : Outport  Port=2
  wires:
  Demux/1 -> L/1
  S-Function/1 -> Demux/1
  Mux/1 -> S-Function/1
  Concentrado/1 -> Mux/1
  Concentracao/1 -> Mux/2
  Agua fresca/1 -> Mux/3
  [FI_111] -> Mux1/1, Mux/4
  Demux/2 -> Mux1/2
  Mux1/1 -> F,C/1

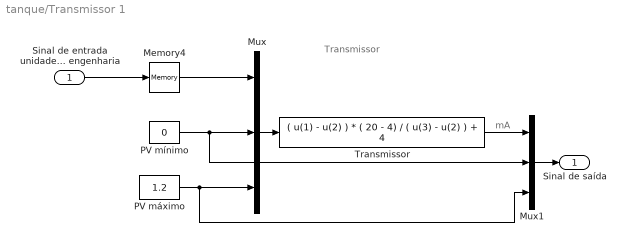
== system tanque/Transmissor 1 ==
  note: mA
  note: Transmissor
  Sinal de entrada unidades de engenharia : Inport
  Memory4 : Memory
  Mux : Mux  Inputs=3
  Mux1 : Mux  Inputs=3
  PV máximo : Constant  Value=1.2
  PV mínimo : Constant  Value=0
  Transmissor : Fcn  Expr=( u(1) - u(2) ) * ( 20 - 4) / ( u(3) - u(2) ) + 4
  Sinal de saída : Outport
  wires:
  Mux/1 -> Transmissor/1
  PV mínimo/1 -> Mux/2, Mux1/2
  PV máximo/1 -> Mux/3, Mux1/3
  Transmissor/1 -> Mux1/1
  Mux1/1 -> Sinal de saída/1
  Sinal de entrada unidades de engenharia/1 -> Memory4/1
  Memory4/1 -> Mux/1

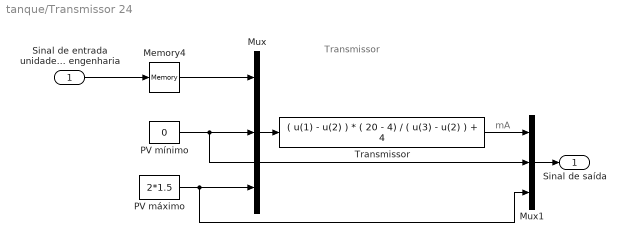
== system tanque/Transmissor 24 ==
  note: mA
  note: Transmissor
  Sinal de entrada unidades de engenharia : Inport
  Memory4 : Memory  X0=0.2
  Mux : Mux  Inputs=3
  Mux1 : Mux  Inputs=3
  PV máximo : Constant  Value=2*1.5
  PV mínimo : Constant  Value=0
  Transmissor : Fcn  Expr=( u(1) - u(2) ) * ( 20 - 4) / ( u(3) - u(2) ) + 4
  Sinal de saída : Outport
  wires:
  Mux/1 -> Transmissor/1
  PV mínimo/1 -> Mux/2, Mux1/2
  PV máximo/1 -> Mux/3, Mux1/3
  Transmissor/1 -> Mux1/1
  Mux1/1 -> Sinal de saída/1
  Sinal de entrada unidades de engenharia/1 -> Memory4/1
  Memory4/1 -> Mux/1

== system tanque/Transmissor 3 ==
  note: Transmissor
  note: mA
  Sinal de entrada unidades de engenharia : Inport
  Mux : Mux  Inputs=3
  Mux1 : Mux  Inputs=3
  PV máximo : Constant  Value=6
  PV mínimo : Constant  Value=0
  Transmissor : Fcn  Expr=( u(1) - u(2) ) * ( 20 - 4) / ( u(3) - u(2) ) + 4
  Sinal de saída : Outport
  wires:
  Mux1/1 -> Sinal de saída/1
  Transmissor/1 -> Mux1/1
  Sinal de entrada unidades de engenharia/1 -> Mux/1
  PV máximo/1 -> Mux1/3, Mux/3
  PV mínimo/1 -> Mux1/2, Mux/2
  Mux/1 -> Transmissor/1

== system tanque/Transmissor 4 ==
  note: Transmissor
  note: mA
  Sinal de entrada unidades de engenharia : Inport
  Memory4 : Memory  X0=1.727
  Mux : Mux  Inputs=3
  Mux1 : Mux  Inputs=3
  PV máximo : Constant  Value=2*4
  PV mínimo : Constant  Value=0
  Transmissor : Fcn  Expr=( u(1) - u(2) ) * ( 20 - 4) / ( u(3) - u(2) ) + 4
  Sinal de saída : Outport
  wires:
  Mux1/1 -> Sinal de saída/1
  Transmissor/1 -> Mux1/1
  Sinal de entrada unidades de engenharia/1 -> Memory4/1
  PV máximo/1 -> Mux1/3, Mux/3
  PV mínimo/1 -> Mux1/2, Mux/2
  Mux/1 -> Transmissor/1
  Memory4/1 -> Mux/1

== system tanque/Transmissor 5 ==
  note: Transmissor
  note: mA
  Sinal de entrada unidades de engenharia : Inport
  Memory : Memory  X0=5.649
  Mux : Mux  Inputs=3
  Mux1 : Mux  Inputs=3
  PV máximo : Constant  Value=0.6
  PV mínimo : Constant  Value=0
  Transmissor : Fcn  Expr=( u(1) - u(2) ) * ( 20 - 4) / ( u(3) - u(2) ) + 4
  Sinal de saída : Outport
  wires:
  Mux1/1 -> Sinal de saída/1
  Transmissor/1 -> Mux1/1
  Sinal de entrada unidades de engenharia/1 -> Memory/1
  PV máximo/1 -> Mux1/3, Mux/3
  PV mínimo/1 -> Mux1/2, Mux/2
  Mux/1 -> Transmissor/1
  Memory/1 -> Mux/1
